simulink model "Lab5_PI_Design"  (R2026a)
settings: Solver=FixedStepDiscrete  StopTime=525  FixedStep=Ts
InitFcn:
  | % Plant model, offsets and pump limits come from ELEC4632_Lab5_SysID.m.
  | % If they are not in the workspace yet, load the saved copy.
  | if ~exist('a1', 'var') || ~exist('umin', 'var')
  |     load(fullfile(fileparts(get_param(bdroot, 'FileName')), 'Lab5_Model.mat'));
  | end
  | % PI gains designed in this model (Part 2). Set Kp / Ki in the workspace
  | % to try other values - the real-time model reads the same two variables.
  | if ~exist('Kp', 'var'), Kp = 1.30; end
  | if ~exist('Ki', 'var'), Ki = 0.045; end
  | fprintf('Lab5_PI_Design: Kp = %.3f, Ki = %.4f, %.2f <= u <= %.2f\n', Kp, Ki, umin, umax);
values from neighbouring files (symbols this model uses):
  a1 = -theta(1)    [ELEC4632_Lab5_SysID.m]    (also in Lab5_Model.mat = -1.37723301589)
  a2 = -theta(2)    [ELEC4632_Lab5_SysID.m]    (also in Lab5_Model.mat = 0.391909364244)
  b1 = theta(3)    [ELEC4632_Lab5_SysID.m]    (also in Lab5_Model.mat = -0.00653030213209)
  b2 = theta(4)    [ELEC4632_Lab5_SysID.m]    (also in Lab5_Model.mat = 0.0509390501561)
  Ts = mean(diff(t_raw))    [ELEC4632_Lab5_SysID.m]    (also in Lab5_Model.mat = 0.75)
  umax = Vmax - u_offset    [ELEC4632_Lab5_SysID.m]    (also in Lab5_Model.mat = 1)
  umin = Vmin - u_offset    [ELEC4632_Lab5_SysID.m]    (also in Lab5_Model.mat = -1)
undefined symbols (not defined in the file or in its folder): Ki, Kp
libraries: slpidlib x1, simulink x1
settings Model: Creator=Jordan Mohindra  LastModifiedBy=Jordan Mohindra

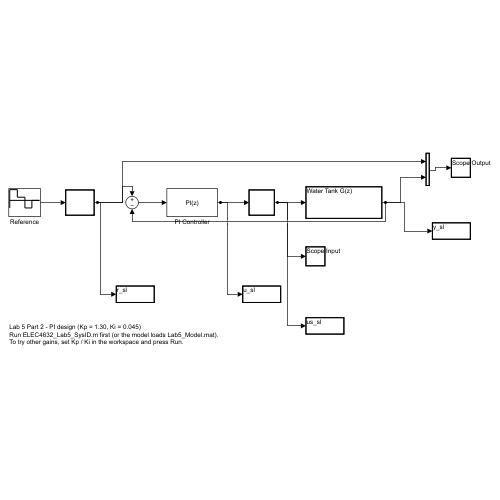
[thumbnail: Simulink's stored preview of the top-level diagram]
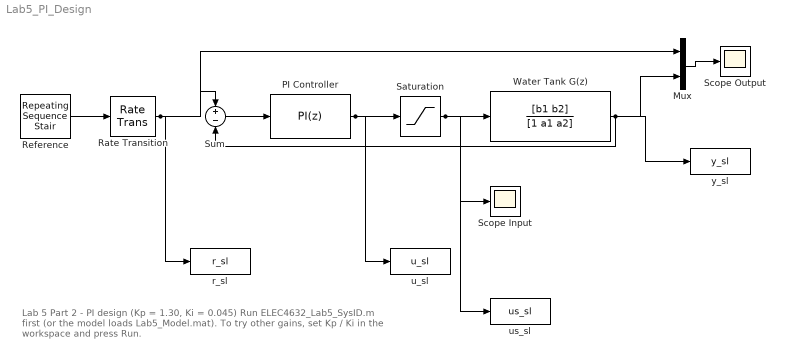
== system Lab5_PI_Design ==
  note: Lab 5 Part 2 - PI design (Kp = 1.30, Ki = 0.045)
      | Run ELEC4632_Lab5_SysID.m first (or the model loads Lab5_Model.mat).
      | To try other gains, set Kp / Ki in the workspace and press Run.
  Mux : Mux  Inputs=2
  PI Controller : slpidlib/PID Controller  Controller=PI  Form=Parallel  TimeDomain=Discrete-time  UseExternalTs=off  SampleTime=Ts  IntegratorMethod=Forward Euler  FilterMethod=Forward Euler  ControllerParametersSource=internal  P=Kp  I=Ki  UseKiTs=off  D=0  UseExternalDerivativeSource=off  N=100  UseFilter=on  TunerSelectOption=Transfer Function Based (PID Tuner App)  InitialConditionSource=internal  InitialConditionForIntegrator=0  InitialConditionForFilter=0  DifferentiatorICPrevScaledInput=0  ExternalReset=none  TrackingMode=off  Kt=1  LimitOutput=off  SatLimitsSource=internal  UpperSaturationLimit=inf  LowerSaturationLimit=-inf  LinearizeAsGain=off  AntiWindupMode=none  Kb=1  LimitIntegrator=off  UpperIntegratorSaturationLimit=inf  LowerIntegratorSaturationLimit=-inf  POutMin=[]  POutMax=[]  IOutMin=[]  IOutMax=[]  DOutMin=[]  DOutMax=[]  NOutMin=[]  NOutMax=[]  SumOutMin=[]  SumOutMax=[]  SaturationOutMin=[]  SaturationOutMax=[]  PParamMin=[]  PParamMax=[]  IParamMin=[]  IParamMax=[]  DParamMin=[]  DParamMax=[]  NParamMin=[]  NParamMax=[]  KbParamMin=[]  KbParamMax=[]  KtParamMin=[]  KtParamMax=[]  KbOutMin=[]  KbOutMax=[]  KtOutMin=[]  KtOutMax=[]  IntegratorOutMin=[]  IntegratorOutMax=[]  FilterOutMin=[]  FilterOutMax=[]  SumI1OutMin=[]  SumI1OutMax=[]  SumI2OutMin=[]  SumI2OutMax=[]  SumI3OutMin=[]  SumI3OutMax=[]  SumI4OutMin=[]  SumI4OutMax=[]  SumDOutMin=[]  SumDOutMax=[]  DifferentiatorOutMin=[]  DifferentiatorOutMax=[]  FilterDiffOutCoefMin=[]  FilterDiffOutCoefMax=[]  ReciprocalOutMin=[]  ReciprocalOutMax=[]  SumDenOutMin=[]  SumDenOutMax=[]  SumNumOutMin=[]  SumNumOutMax=[]  DivideOutMin=[]  DivideOutMax=[]  UdiffTsProdOutMin=[]  UdiffTsProdOutMax=[]  NTsProdOutMin=[]  NTsProdOutMax=[]  UintegralTsProdOutMin=[]  UintegralTsProdOutMax=[]  UngainTsProdOutMin=[]  UngainTsProdOutMax=[]  ClampingZeroOutDataTypeStr=Inherit: Inherit via back propagation  ClampingZeroOutMin=[]  ClampingZeroOutMax=[]  FilterDenConstantOutDataTypeStr=Inherit: Inherit via back propagation  FilterDenConstantOutMin=[]  FilterDenConstantOutMax=[]  PCopyOutDataTypeStr=Inherit: Inherit via back propagation  PCopyOutMin=[]  PCopyOutMax=[]  NCopyOutDataTypeStr=Inherit: Inherit via back propagation  NCopyOutMin=[]  NCopyOutMax=[]  IntegratorContinuousStateAttributes=''  IntegratorStateMustResolveToSignalObject=off  IntegratorRTWStateStorageClass=Auto  FilterContinuousStateAttributes=''  FilterStateMustResolveToSignalObject=off  FilterRTWStateStorageClass=Auto  ParallelPVariant=InternalParameters  IdealPVariant=Disabled  IVariant=InternalParameters  DVariant=Disabled  IntegratorVariant=Discrete  SatVariant=Disabled  AWVariant=Passthrough  PCopyVariant=Disabled  TRVariant=Disabled  FdbkBlocksVariant=Forward  IdealPFdbkVariant=Disabled  SatFdbkVariant=Disabled  DerivativeFilterVariant=Disabled  NVariant=Disabled  NCopyVariant=Disabled_SignalSpec  FilterICVariant=Disabled  IntegratorICVariant=InternalICs  ExternalResetVariant=Disabled  TRSumVariant=Passthrough  SumFdbkVariant=Disabled  SumVariant=Sum_PI  TsampFilterVariant=InternalTs  TsampNgainVariant=Passthrough  TsampIntegralVariant=Disabled_SignalSpec  ExternalSaturationOutDataTypeStr=Inherit: Same as second input  DerivativeSourceVariant=Disabled  PreIntVariant=InternalPreInt
      settings: LibrarySourceBlock=simulink/Discrete/Discrete PID Controller
  Rate Transition : RateTransition  OutPortSampleTime=Ts
  Reference : simulink/Sources/Repeating Sequence Stair  OutValues=[0.7;0.2;-0.5;0]  tsamp=140*Ts  OutMin=[]  OutMax=[]  OutDataTypeStr=double  OutputDataTypeScalingMode=double  OutDataType=fixdt(0,8)  ConRadixGroup=Best Precision: Vector-wise  OutScaling=2^-12
  Saturation : Saturate  UpperLimit=umax  LowerLimit=umin
  Scope Input : Scope
  Scope Output : Scope
  Sum : Sum  Inputs=+-
  Water Tank G(z) : DiscreteTransferFcn  Numerator=[b1 b2]  Denominator=[1 a1 a2]  SampleTime=Ts
  r_sl : ToWorkspace  VariableName=r_sl  SampleTime=-1
  u_sl : ToWorkspace  VariableName=u_sl  SampleTime=-1
  us_sl : ToWorkspace  VariableName=us_sl  SampleTime=-1
  y_sl : ToWorkspace  VariableName=y_sl  SampleTime=-1
  wires:
  Reference/1 -> Rate Transition/1
  Rate Transition/1 -> Sum/1, Mux/1, r_sl/1
  Sum/1 -> PI Controller/1
  PI Controller/1 -> Saturation/1, u_sl/1
  Saturation/1 -> Water Tank G(z)/1, Scope Input/1, us_sl/1
  Water Tank G(z)/1 -> Sum/2, Mux/2, y_sl/1
  Mux/1 -> Scope Output/1
